simulink model "Finalannfaultdetecandclass"  (R2024b)
settings: Solver=ode45  StartTime=0.0  StopTime=0.4  FixedStep=1e-6  MaxStep=0.04  RelTol=1e-3  EnableMultiTasking=on
PreLoadFcn:
  | power_13NodeTestFeeder_init;
values from neighbouring files (symbols this model uses):
  C_601 = [1.03835973183e-08  -3.28956213337e-09  -2.07596127216e-09; -3.28956213337e-09  9.8230300863e-09  -1.22250137004e-09; -2.07596127216e-09  -1.22250137004e-09  9.29377945947e-09]    [Finalmat.mat]    (also in bus1.mat; bus10.mat; bus11.mat; bus12.mat)
  C_602 = [9.39333329896e-09  -1.78290377777e-09  -2.78635373607e-09; -1.78290377777e-09  8.5370713848e-09  -1.08586207709e-09; -2.78635373607e-09  -1.08586207709e-09  8.94105559107e-09]    [Finalmat.mat]    (also in bus1.mat; bus10.mat; bus11.mat; bus12.mat)
  C_603 = [0  0  0; 0  7.76272711671e-09  -1.48325331387e-09; 0  -1.48325331387e-09  7.69036927641e-09]    [Finalmat.mat]    (also in bus1.mat; bus10.mat; bus11.mat; bus12.mat)
  C_604 = [7.69036927641e-09  0  -1.48325331387e-09; 0  0  0; -1.48325331387e-09  0  7.76272711671e-09]    [Finalmat.mat]    (also in bus1.mat; bus10.mat; bus11.mat; bus12.mat)
  C_605 = [0  0  0; 0  0  0; 0  0  7.44890176838e-09]    [Finalmat.mat]    (also in bus1.mat; bus10.mat; bus11.mat; bus12.mat)
  C_606 = [1.59697709306e-07  -1.64824237567e-15  -1.64824237567e-15; -1.64824237567e-15  1.59697709306e-07  -1.64824237567e-15; -1.64824237567e-15  -1.64824237567e-15  1.59697709306e-07]    [Finalmat.mat]    (also in bus1.mat; bus10.mat; bus11.mat; bus12.mat)
  C_607 = [1.46679066902e-07  0  0; 0  0  0; 0  0  0]    [Finalmat.mat]    (also in bus1.mat; bus10.mat; bus11.mat; bus12.mat)
  ft2km = 0.0003048    [Finalmat.mat]    (also in bus1.mat; bus10.mat; bus11.mat; bus12.mat)
  L_601 = [0.0016777459142  0.000826923199875  0.000698195470335; 0.000826923199875  0.00172702836123  0.000634408490396; 0.000698195470335  0.000634408490396  0.00170560121035]    [Finalmat.mat]    (also in bus1.mat; bus10.mat; bus11.mat; bus12.mat)
  L_602 = [0.00194723354262  0.000698195470335  0.000826923199875; 0.000698195470335  0.00197508883877  0.000634408490396; 0.000826923199875  0.000634408490396  0.00199635116541]    [Finalmat.mat]    (also in bus1.mat; bus10.mat; bus11.mat; bus12.mat)
  L_603 = [0  0  0; 0  0.00222034730427  0.000756708074671; 0  0.000756708074671  0.00223650007955]    [Finalmat.mat]    (also in bus1.mat; bus10.mat; bus11.mat; bus12.mat)
  L_604 = [0.00223650007955  0  0.000756708074671; 0  0  0; 0.000756708074671  0  0.00222034730427]    [Finalmat.mat]    (also in bus1.mat; bus10.mat; bus11.mat; bus12.mat)
  L_605 = [0  0  0; 0  0  0; 0  0  0.00222100660122]    [Finalmat.mat]    (also in bus1.mat; bus10.mat; bus11.mat; bus12.mat)
  L_606 = [0.000735610572263  5.40623499221e-05  2.35698659721e-05; 5.40623499221e-05  0.000666054744009  5.40623499221e-05; 2.35698659721e-05  5.40623499221e-05  0.000735610572263]    [Finalmat.mat]    (also in bus1.mat; bus10.mat; bus11.mat; bus12.mat)
  L_607 = [0.000844559393295  0  0; 0  0  0; 0  0  0]    [Finalmat.mat]    (also in bus1.mat; bus10.mat; bus11.mat; bus12.mat)
  R_601 = [0.215305653249  0.0969341469174  0.0981768923907; 0.0969341469174  0.209713298619  0.0953807150757; 0.0981768923907  0.0953807150757  0.212136652292]    [Finalmat.mat]    (also in bus1.mat; bus10.mat; bus11.mat; bus12.mat)
  R_602 = [0.467645121603  0.0981768923907  0.0969341469174; 0.0981768923907  0.464476120646  0.0953807150757; 0.0969341469174  0.0953807150757  0.462052766973]    [Finalmat.mat]    (also in bus1.mat; bus10.mat; bus11.mat; bus12.mat)
  R_603 = [0  0  0; 0  0.826052916102  0.128375607392; 0  0.128375607392  0.822573228777]    [Finalmat.mat]    (also in bus1.mat; bus10.mat; bus11.mat; bus12.mat)
  R_604 = [0.822573228777  0  0.128375607392; 0  0  0; 0.128375607392  0  0.826052916102]    [Finalmat.mat]    (also in bus1.mat; bus10.mat; bus11.mat; bus12.mat)
  R_605 = [0  0  0; 0  0  0; 0  0  0.825928641555]    [Finalmat.mat]    (also in bus1.mat; bus10.mat; bus11.mat; bus12.mat)
  R_606 = [0.495979718394  0.198342177539  0.177029092672; 0.198342177539  0.49032522649  0.198342177539; 0.177029092672  0.198342177539  0.495979718394]    [Finalmat.mat]    (also in bus1.mat; bus10.mat; bus11.mat; bus12.mat)
  R_607 = [0.834192898952  0  0; 0  0  0; 0  0  0]    [Finalmat.mat]    (also in bus1.mat; bus10.mat; bus11.mat; bus12.mat)
libraries: neural x123, spsLoadFlowBusLib x12, spsDistributedParametersLineLib x9, spsThreePhaseSeriesRLCLoadLib x7, spsMultimeterLib x6, spsPowerPhasorLib x6, spsSeriesRLCLoadLib x5, spsThreePhaseVIMeasurementLib x4, spsGroundLib x4, spsThreePhaseSourceLib x1, spsThreePhaseBreakerLib x1, simulink x1
(part 4 of 4)

== system Finalannfaultdetecandclass/Subsystem1/Function Fitting Neural Network/Layer 2/Delays 1 ==
  "p{2}" : Inport  PortDimensions=100
      mask Display: e = 0.06;c1 = [120 230 180]/255;c2 = ([120 230 180]+0)/(256+128);c3 = ([120 230 180]+128)/(256+128);patch([0 1 1 0],[0 0 1 1],c1);patch([0 1 1 1-e 1-e 0+e],[0 0 1 1-e 0+e 0+e],c2);patch([0 0 1 1-e 0+e 0+e],[0 1 1 1-e 1-e 0+e],c3);plot([0 1 1 0 0],[0 0 1 1 0]);
  mux : Mux  Inputs=1
      mask Display: e = 0.06;c1 = [120 150 230]/255;c2 = ([120 150 230]+0)/383;c3 = ([120 150 230]+128)/383;patch([0 1 1 0],[0 0 1 1],c1);patch([0 1 1 1-e 1-e 0+e],[0 0 1 1-e 0+e 0+e],c2);patch([0 0 1 1-e 0+e 0+e],[0 1 1 1-e 1-e 0+e],c3);plot([0 1 1 0 0],[0 0 1 1 0]);disp('Mux')
  "pd{2,1}" : Outport
      mask Display: e = 0.06;c1 = [120 230 180]/255;c2 = ([120 230 180]+0)/(256+128);c3 = ([120 230 180]+128)/(256+128);patch([0 1 1 0],[0 0 1 1],c1);patch([0 1 1 1-e 1-e 0+e],[0 0 1 1-e 0+e 0+e],c2);patch([0 0 1 1-e 0+e 0+e],[0 1 1 1-e 1-e 0+e],c3);plot([0 1 1 0 0],[0 0 1 1 0]);
  wires:
  "p{2}"/1 -> mux/1
  mux/1 -> "pd{2,1}"/1

== system Finalannfaultdetecandclass/Subsystem1/Function Fitting Neural Network/Layer 2/LW{2,1} ==
  "ad{2,1}" : Inport  PortDimensions=100
      mask Display: e = 0.06;c1 = [120 230 180]/255;c2 = ([120 230 180]+0)/(256+128);c3 = ([120 230 180]+128)/(256+128);patch([0 1 1 0],[0 0 1 1],c1);patch([0 1 1 1-e 1-e 0+e],[0 0 1 1-e 0+e 0+e],c2);patch([0 0 1 1-e 0+e 0+e],[0 1 1 1-e 1-e 0+e],c3);plot([0 1 1 0 0],[0 0 1 1 0]);
  "IW{2,1}(1,:)'" : Constant  Value=[1.8793908287279783575485225810552947223186492919921875;-0.9048667518245905316831567688495852053165435791015625;-0.92458538808867185565532054170034825801849365234375;-2.02532521067546245063795140595175325870513916015625;5.33525657670273556476558951544575393199920654296875;3.210800612231773154547909143730066716670989990234375;-0.09324484938112427567791229421345633454620838165283203125;0.03540388689183378290170622904042829759418964385986328125;0.1885587765727710640728531643617316149175167083740234375;-4.22107099118371120738402169081382453441619873046875;-0.264501726010362647745211006622412241995334625244140625;-0.34225779722053040199369888796354644000530242919921875;-0.373202417779953388166092054234468378126621246337890625;8.2600182662194896465734927915036678314208984375;-3.2632258813898840088540964643470942974090576171875;-0.62922711116860108315762545316829346120357513427734375;-0.38755461469218255299296060911729000508785247802734375;0.65203344442902988475907477550208568572998046875;-2.26821878466440285393446174566633999347686767578125;0.543177487170682926631570808240212500095367431640625;-2.789913530456374690658094550599344074726104736328125;0.1798698221775162642277479108088300563395023345947265625;0.399305983587987689542586622337694279849529266357421875;1.2306887105144139749057785593322478234767913818359375;1.456708317179773448657442713738419115543365478515625;1.035561461053104093110732719651423394680023193359375;0.27441751827051164003279382086475379765033721923828125;-0.204970973074732831786803899376536719501018524169921875;-0.253112822104407164669481744567747227847576141357421875;0.1510518587617716013138391417669481597840785980224609375;-0.31745069317599250435790736446506343781948089599609375;-0.676791919103845618366221970063634216785430908203125;-2.978627056642336068392751258215866982936859130859375;9.0535751730324189878729157499037683010101318359375;-8.190932561555936075592398992739617824554443359375;0.49841770298888565804418249172158539295196533203125;-0.50061513193962159373739950751769356429576873779296875;1.53295551447780287190880699199624359607696533203125;12.583976878439415258981171064078807830810546875;-0.09178682720573481945702809525755583308637142181396484375;8.636594135212391165623557753860950469970703125;3.910230596444252970655952594825066626071929931640625;-2.50969331155198016602980715106241405010223388671875;-0.32572264372845494140307209818274714052677154541015625;2.658418596062821048775504095829091966152191162109375;4.26885657500254556140362183214165270328521728515625;1.4483077928253802468816502369008958339691162109375;-1.0548868080331390562065507765510119497776031494140625;-1.75700921521880726317021981230936944484710693359375;-4.8518766072740096007009924505837261676788330078125;-0.043810031439321835133871019252183032222092151641845703125;0.418247245768505415686178139367257244884967803955078125;-1.54235777001860352442008661455474793910980224609375;0.2440732320832143809052894312117132358253002166748046875;-2.981478415506142010116263918462209403514862060546875;-0.1983812993079519804151544803971773944795131683349609375;-0.488626450603534212557832461243378929793834686279296875;-4.16709607961305028567267072503454983234405517578125;2.59533520027240083294373107491992413997650146484375;4.20601887646172389878529429552145302295684814453125;3.531120270555935025669214155641384422779083251953125;-0.51904717173316872180777181711164303123950958251953125;1.751606913577048896257792875985614955425262451171875;2.297924274586310655621446130680851638317108154296875;0.10235191318978331675992876625969074666500091552734375;0.68318748611821000782384771810029633343219757080078125;1.0577758447114204987116181655437685549259185791015625;3.15370331022145489185959377209655940532684326171875;1.325141327935329460530056167044676840305328369140625;4.03421651104892742267793437349610030651092529296875;-9.5505906993198106391673718462698161602020263671875;-0.21252767811685158161338904392323456704616546630859375 ...(+1553 chars)]
      mask Display: e = 0.06;c1 = [120 150 230]/255;c2 = ([120 150 230]+0)/383;c3 = ([120 150 230]+128)/383;patch([0 1 1 0],[0 0 1 1],c1);patch([0 1 1 1-e 1-e 0+e],[0 0 1 1-e 0+e 0+e],c2);patch([0 0 1 1-e 0+e 0+e],[0 1 1 1-e 1-e 0+e],c3);plot([0 1 1 0 0],[0 0 1 1 0]);disp('weights');
  Mux : Mux  Inputs=1
      mask Display: e = 0.06;c1 = [120 150 230]/255;c2 = ([120 150 230]+0)/383;c3 = ([120 150 230]+128)/383;patch([0 1 1 0],[0 0 1 1],c1);patch([0 1 1 1-e 1-e 0+e],[0 0 1 1-e 0+e 0+e],c2);patch([0 0 1 1-e 0+e 0+e],[0 1 1 1-e 1-e 0+e],c3);plot([0 1 1 0 0],[0 0 1 1 0]);disp('Mux');
  dotprod1 : neural/Weight Functions/dotprod
  "lz{2,1}" : Outport
      mask Display: e = 0.06;c1 = [120 230 180]/255;c2 = ([120 230 180]+0)/(256+128);c3 = ([120 230 180]+128)/(256+128);patch([0 1 1 0],[0 0 1 1],c1);patch([0 1 1 1-e 1-e 0+e],[0 0 1 1-e 0+e 0+e],c2);patch([0 0 1 1-e 0+e 0+e],[0 1 1 1-e 1-e 0+e],c3);plot([0 1 1 0 0],[0 0 1 1 0]);
  wires:
  "IW{2,1}(1,:)'"/1 -> dotprod1/1
  "ad{2,1}"/1 -> dotprod1/2
  dotprod1/1 -> Mux/1
  Mux/1 -> "lz{2,1}"/1

== system Finalannfaultdetecandclass/Subsystem1/Function Fitting Neural Network1/Layer 1/Delays 1 ==
  "p{1}" : Inport  PortDimensions=9
      mask Display: e = 0.06;c1 = [120 230 180]/255;c2 = ([120 230 180]+0)/(256+128);c3 = ([120 230 180]+128)/(256+128);patch([0 1 1 0],[0 0 1 1],c1);patch([0 1 1 1-e 1-e 0+e],[0 0 1 1-e 0+e 0+e],c2);patch([0 0 1 1-e 0+e 0+e],[0 1 1 1-e 1-e 0+e],c3);plot([0 1 1 0 0],[0 0 1 1 0]);
  mux : Mux  Inputs=1
      mask Display: e = 0.06;c1 = [120 150 230]/255;c2 = ([120 150 230]+0)/383;c3 = ([120 150 230]+128)/383;patch([0 1 1 0],[0 0 1 1],c1);patch([0 1 1 1-e 1-e 0+e],[0 0 1 1-e 0+e 0+e],c2);patch([0 0 1 1-e 0+e 0+e],[0 1 1 1-e 1-e 0+e],c3);plot([0 1 1 0 0],[0 0 1 1 0]);disp('Mux')
  "pd{1,1}" : Outport
      mask Display: e = 0.06;c1 = [120 230 180]/255;c2 = ([120 230 180]+0)/(256+128);c3 = ([120 230 180]+128)/(256+128);patch([0 1 1 0],[0 0 1 1],c1);patch([0 1 1 1-e 1-e 0+e],[0 0 1 1-e 0+e 0+e],c2);patch([0 0 1 1-e 0+e 0+e],[0 1 1 1-e 1-e 0+e],c3);plot([0 1 1 0 0],[0 0 1 1 0]);
  wires:
  "p{1}"/1 -> mux/1
  mux/1 -> "pd{1,1}"/1

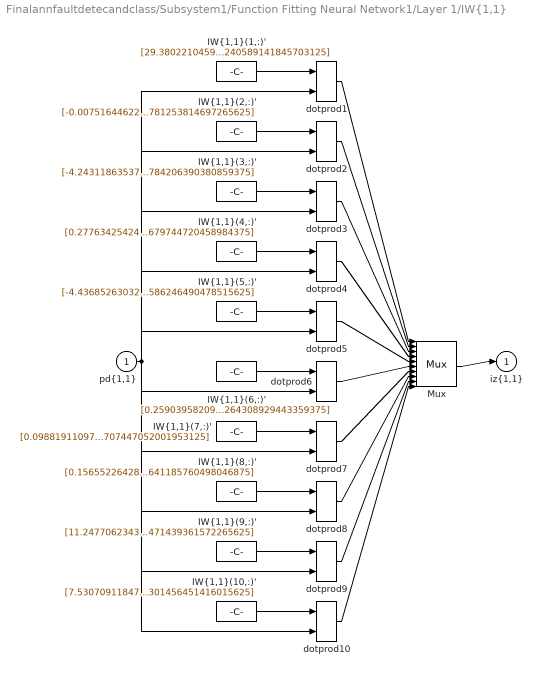
== system Finalannfaultdetecandclass/Subsystem1/Function Fitting Neural Network1/Layer 1/IW{1,1} ==
  "pd{1,1}" : Inport  PortDimensions=9
      mask Display: e = 0.06;c1 = [120 230 180]/255;c2 = ([120 230 180]+0)/(256+128);c3 = ([120 230 180]+128)/(256+128);patch([0 1 1 0],[0 0 1 1],c1);patch([0 1 1 1-e 1-e 0+e],[0 0 1 1-e 0+e 0+e],c2);patch([0 0 1 1-e 0+e 0+e],[0 1 1 1-e 1-e 0+e],c3);plot([0 1 1 0 0],[0 0 1 1 0]);
  "IW{1,1}(1,:)'" : Constant  Value=[29.38022104594626426887771231122314929962158203125;-1.583758512931292106173941647284664213657379150390625;-12.887641563029934133055576239712536334991455078125;15.3742096899572491253138650790788233280181884765625;-0.452999735082487919868299286463297903537750244140625;-11.2742404077810487450506116147153079509735107421875;0.253929560001421028569978943778551183640956878662109375;13.720895642811651526926652877591550350189208984375;3.625389934006417735901095511508174240589141845703125]
      mask Display: e = 0.06;c1 = [120 150 230]/255;c2 = ([120 150 230]+0)/383;c3 = ([120 150 230]+128)/383;patch([0 1 1 0],[0 0 1 1],c1);patch([0 1 1 1-e 1-e 0+e],[0 0 1 1-e 0+e 0+e],c2);patch([0 0 1 1-e 0+e 0+e],[0 1 1 1-e 1-e 0+e],c3);plot([0 1 1 0 0],[0 0 1 1 0]);disp('Weights');
  "IW{1,1}(10,:)'" : Constant  Value=[7.530709118478295494014673749916255474090576171875;6.41481450944031461602889976347796618938446044921875;5.7414808644690840111479701590724289417266845703125;-1.0144361351505650770121746973018161952495574951171875;0.60391139595748588586587857207632623612880706787109375;0.175120384899493497510292172592016868293285369873046875;-6.341914830455859686253461404703557491302490234375;1.329104495916630934715385592426173388957977294921875;4.685489713819865897903582663275301456451416015625]
      mask Display: e = 0.06;c1 = [120 150 230]/255;c2 = ([120 150 230]+0)/383;c3 = ([120 150 230]+128)/383;patch([0 1 1 0],[0 0 1 1],c1);patch([0 1 1 1-e 1-e 0+e],[0 0 1 1-e 0+e 0+e],c2);patch([0 0 1 1-e 0+e 0+e],[0 1 1 1-e 1-e 0+e],c3);plot([0 1 1 0 0],[0 0 1 1 0]);disp('Weights');
  "IW{1,1}(2,:)'" : Constant  Value=[-0.007516446226203031544255139806409715674817562103271484375;-0.052171455998463005243603873850588570348918437957763671875;40.07240766673493226335267536342144012451171875;-0.529361813414303217228962239460088312625885009765625;-0.1313103612760208316334598066532635129988193511962890625;0.492305801062109138488409598721773363649845123291015625;-0.2409650475170437566863057554655824787914752960205078125;-9.543939777753767117474126280285418033599853515625;9.0870090560286005398893394158221781253814697265625]
      mask Display: e = 0.06;c1 = [120 150 230]/255;c2 = ([120 150 230]+0)/383;c3 = ([120 150 230]+128)/383;patch([0 1 1 0],[0 0 1 1],c1);patch([0 1 1 1-e 1-e 0+e],[0 0 1 1-e 0+e 0+e],c2);patch([0 0 1 1-e 0+e 0+e],[0 1 1 1-e 1-e 0+e],c3);plot([0 1 1 0 0],[0 0 1 1 0]);disp('Weights');
  "IW{1,1}(3,:)'" : Constant  Value=[-4.24311863537578748406531303771771490573883056640625;-0.56605455006675431395279929347452707588672637939453125;7.69263762371459502986681400216184556484222412109375;-0.2345349318144732964075416248306282795965671539306640625;0.43859983264558854987313907258794642984867095947265625;0.72900485968290917870859857430332340300083160400390625;-0.6106674688833038100455041785608045756816864013671875;-1.4125342046991329336691478602006100118160247802734375;0.954529878403048481771975275478325784206390380859375]
      mask Display: e = 0.06;c1 = [120 150 230]/255;c2 = ([120 150 230]+0)/383;c3 = ([120 150 230]+128)/383;patch([0 1 1 0],[0 0 1 1],c1);patch([0 1 1 1-e 1-e 0+e],[0 0 1 1-e 0+e 0+e],c2);patch([0 0 1 1-e 0+e 0+e],[0 1 1 1-e 1-e 0+e],c3);plot([0 1 1 0 0],[0 0 1 1 0]);disp('Weights');
  "IW{1,1}(4,:)'" : Constant  Value=[0.27763425424716647871292707350221462547779083251953125;-3.3827539479368713415396996424533426761627197265625;-0.487081651909694601787492729272344149649143218994140625;-6.9426781475629635309587683877907693386077880859375;0.2001253526836813956268912306768470443785190582275390625;-0.321497490473505731500836191116832196712493896484375;-12.4322080410378870141130391857586801052093505859375;12.5879994895972320279042833135463297367095947265625;0.27710769892183806373253673882572911679744720458984375]
      mask Display: e = 0.06;c1 = [120 150 230]/255;c2 = ([120 150 230]+0)/383;c3 = ([120 150 230]+128)/383;patch([0 1 1 0],[0 0 1 1],c1);patch([0 1 1 1-e 1-e 0+e],[0 0 1 1-e 0+e 0+e],c2);patch([0 0 1 1-e 0+e 0+e],[0 1 1 1-e 1-e 0+e],c3);plot([0 1 1 0 0],[0 0 1 1 0]);disp('Weights');
  "IW{1,1}(5,:)'" : Constant  Value=[-4.4368526303241448971448335214518010616302490234375;-3.593845053872443795484059592126868665218353271484375;10.1550055068302498284538160078227519989013671875;-0.49914763675904272322014776364085264503955841064453125;0.5660702345538994872953253434388898313045501708984375;1.37378804025246825659678506781347095966339111328125;-0.405236667080652368522208917056559585034847259521484375;-1.4087649953617231712854618308483622968196868896484375;1.5632128167424907960736391032696701586246490478515625]
      mask Display: e = 0.06;c1 = [120 150 230]/255;c2 = ([120 150 230]+0)/383;c3 = ([120 150 230]+128)/383;patch([0 1 1 0],[0 0 1 1],c1);patch([0 1 1 1-e 1-e 0+e],[0 0 1 1-e 0+e 0+e],c2);patch([0 0 1 1-e 0+e 0+e],[0 1 1 1-e 1-e 0+e],c3);plot([0 1 1 0 0],[0 0 1 1 0]);disp('Weights');
  "IW{1,1}(6,:)'" : Constant  Value=[0.25903958209407884627495377571904100477695465087890625;-14.1728596158761632750611170195043087005615234375;13.9842637333953359046745390514843165874481201171875;-0.18984682930795060418205366659094579517841339111328125;-0.3858122437420750117098577902652323246002197265625;0.66984843931265292127363863983191549777984619140625;-4.72065980238203319885315067949704825878143310546875;5.22961841369345581398420108598656952381134033203125;3.5168686234222885644840062013827264308929443359375]
      mask Display: e = 0.06;c1 = [120 150 230]/255;c2 = ([120 150 230]+0)/383;c3 = ([120 150 230]+128)/383;patch([0 1 1 0],[0 0 1 1],c1);patch([0 1 1 1-e 1-e 0+e],[0 0 1 1-e 0+e 0+e],c2);patch([0 0 1 1-e 0+e 0+e],[0 1 1 1-e 1-e 0+e],c3);plot([0 1 1 0 0],[0 0 1 1 0]);disp('Weights');
  "IW{1,1}(7,:)'" : Constant  Value=[0.0988191109786849819496268310103914700448513031005859375;29.522862844008496807646224624477326869964599609375;0.4973642899908086167926057896693237125873565673828125;-7.157403678754118203642065054737031459808349609375;9.3605112948433220054766934481449425220489501953125;-0.4133008665678818971400687587447464466094970703125;-22.339928592137457741273465217091143131256103515625;-4.193358410228416488507718895561993122100830078125;-2.057182487229031853104288529721088707447052001953125]
      mask Display: e = 0.06;c1 = [120 150 230]/255;c2 = ([120 150 230]+0)/383;c3 = ([120 150 230]+128)/383;patch([0 1 1 0],[0 0 1 1],c1);patch([0 1 1 1-e 1-e 0+e],[0 0 1 1-e 0+e 0+e],c2);patch([0 0 1 1-e 0+e 0+e],[0 1 1 1-e 1-e 0+e],c3);plot([0 1 1 0 0],[0 0 1 1 0]);disp('Weights');
  "IW{1,1}(8,:)'" : Constant  Value=[0.1565522642874812297986153453166480176150798797607421875;0.07335552424086433376260174554772675037384033203125;0.493599606767612775204412400853470899164676666259765625;-2.575576222935119563572925471817143261432647705078125;-5.204489703361520724911315483041107654571533203125;-1.495166781266143107842481185798533260822296142578125;-0.30736378638011974118171565351076424121856689453125;-24.3238565177839376474366872571408748626708984375;0.9721005384518004444061034519108943641185760498046875]
      mask Display: e = 0.06;c1 = [120 150 230]/255;c2 = ([120 150 230]+0)/383;c3 = ([120 150 230]+128)/383;patch([0 1 1 0],[0 0 1 1],c1);patch([0 1 1 1-e 1-e 0+e],[0 0 1 1-e 0+e 0+e],c2);patch([0 0 1 1-e 0+e 0+e],[0 1 1 1-e 1-e 0+e],c3);plot([0 1 1 0 0],[0 0 1 1 0]);disp('Weights');
  "IW{1,1}(9,:)'" : Constant  Value=[11.2477062343173290770437233732081949710845947265625;0.01906889569289538233221037444309331476688385009765625;3.306004742964588682951898590545170009136199951171875;-0.4465209024047254171563281488488428294658660888671875;-0.154686319042484476948828842068905942142009735107421875;-0.039328003291225162307842566633553360588848590850830078125;0.1089866231528095752434381893181125633418560028076171875;-6.49190528631474439436033208039589226245880126953125;5.89332989152609432181861848221160471439361572265625]
      mask Display: e = 0.06;c1 = [120 150 230]/255;c2 = ([120 150 230]+0)/383;c3 = ([120 150 230]+128)/383;patch([0 1 1 0],[0 0 1 1],c1);patch([0 1 1 1-e 1-e 0+e],[0 0 1 1-e 0+e 0+e],c2);patch([0 0 1 1-e 0+e 0+e],[0 1 1 1-e 1-e 0+e],c3);plot([0 1 1 0 0],[0 0 1 1 0]);disp('Weights');
  Mux : Mux  Inputs=10
      mask Display: e = 0.06;c1 = [120 150 230]/255;c2 = ([120 150 230]+0)/383;c3 = ([120 150 230]+128)/383;patch([0 1 1 0],[0 0 1 1],c1);patch([0 1 1 1-e 1-e 0+e],[0 0 1 1-e 0+e 0+e],c2);patch([0 0 1 1-e 0+e 0+e],[0 1 1 1-e 1-e 0+e],c3);plot([0 1 1 0 0],[0 0 1 1 0]);disp('Mux');
  dotprod{1..10} (10 alike) : neural/Weight Functions/dotprod
  "iz{1,1}" : Outport
      mask Display: e = 0.06;c1 = [120 230 180]/255;c2 = ([120 230 180]+0)/(256+128);c3 = ([120 230 180]+128)/(256+128);patch([0 1 1 0],[0 0 1 1],c1);patch([0 1 1 1-e 1-e 0+e],[0 0 1 1-e 0+e 0+e],c2);patch([0 0 1 1-e 0+e 0+e],[0 1 1 1-e 1-e 0+e],c3);plot([0 1 1 0 0],[0 0 1 1 0]);
  wires:
  "IW{1,1}(1,:)'"/1 -> dotprod1/1
  "pd{1,1}"/1 -> dotprod1/2, dotprod2/2, dotprod3/2, dotprod4/2, dotprod5/2, dotprod6/2, dotprod7/2, dotprod8/2, dotprod9/2, dotprod10/2
  dotprod1/1 -> Mux/1
  "IW{1,1}(2,:)'"/1 -> dotprod2/1
  dotprod2/1 -> Mux/2
  "IW{1,1}(3,:)'"/1 -> dotprod3/1
  dotprod3/1 -> Mux/3
  "IW{1,1}(4,:)'"/1 -> dotprod4/1
  dotprod4/1 -> Mux/4
  "IW{1,1}(5,:)'"/1 -> dotprod5/1
  dotprod5/1 -> Mux/5
  "IW{1,1}(6,:)'"/1 -> dotprod6/1
  dotprod6/1 -> Mux/6
  "IW{1,1}(7,:)'"/1 -> dotprod7/1
  dotprod7/1 -> Mux/7
  "IW{1,1}(8,:)'"/1 -> dotprod8/1
  dotprod8/1 -> Mux/8
  "IW{1,1}(9,:)'"/1 -> dotprod9/1
  dotprod9/1 -> Mux/9
  "IW{1,1}(10,:)'"/1 -> dotprod10/1
  dotprod10/1 -> Mux/10
  Mux/1 -> "iz{1,1}"/1

== system Finalannfaultdetecandclass/Subsystem1/Function Fitting Neural Network1/Layer 2/Delays 1 ==
  "p{2}" : Inport  PortDimensions=10
      mask Display: e = 0.06;c1 = [120 230 180]/255;c2 = ([120 230 180]+0)/(256+128);c3 = ([120 230 180]+128)/(256+128);patch([0 1 1 0],[0 0 1 1],c1);patch([0 1 1 1-e 1-e 0+e],[0 0 1 1-e 0+e 0+e],c2);patch([0 0 1 1-e 0+e 0+e],[0 1 1 1-e 1-e 0+e],c3);plot([0 1 1 0 0],[0 0 1 1 0]);
  mux : Mux  Inputs=1
      mask Display: e = 0.06;c1 = [120 150 230]/255;c2 = ([120 150 230]+0)/383;c3 = ([120 150 230]+128)/383;patch([0 1 1 0],[0 0 1 1],c1);patch([0 1 1 1-e 1-e 0+e],[0 0 1 1-e 0+e 0+e],c2);patch([0 0 1 1-e 0+e 0+e],[0 1 1 1-e 1-e 0+e],c3);plot([0 1 1 0 0],[0 0 1 1 0]);disp('Mux')
  "pd{2,1}" : Outport
      mask Display: e = 0.06;c1 = [120 230 180]/255;c2 = ([120 230 180]+0)/(256+128);c3 = ([120 230 180]+128)/(256+128);patch([0 1 1 0],[0 0 1 1],c1);patch([0 1 1 1-e 1-e 0+e],[0 0 1 1-e 0+e 0+e],c2);patch([0 0 1 1-e 0+e 0+e],[0 1 1 1-e 1-e 0+e],c3);plot([0 1 1 0 0],[0 0 1 1 0]);
  wires:
  "p{2}"/1 -> mux/1
  mux/1 -> "pd{2,1}"/1

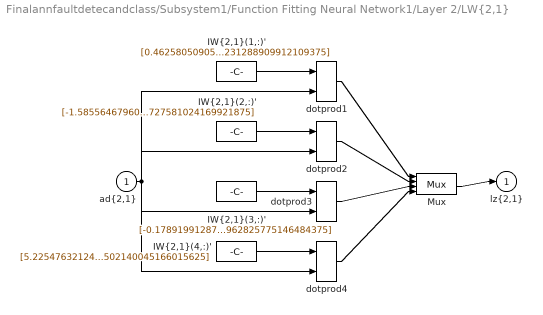
== system Finalannfaultdetecandclass/Subsystem1/Function Fitting Neural Network1/Layer 2/LW{2,1} ==
  "ad{2,1}" : Inport  PortDimensions=10
      mask Display: e = 0.06;c1 = [120 230 180]/255;c2 = ([120 230 180]+0)/(256+128);c3 = ([120 230 180]+128)/(256+128);patch([0 1 1 0],[0 0 1 1],c1);patch([0 1 1 1-e 1-e 0+e],[0 0 1 1-e 0+e 0+e],c2);patch([0 0 1 1-e 0+e 0+e],[0 1 1 1-e 1-e 0+e],c3);plot([0 1 1 0 0],[0 0 1 1 0]);
  "IW{2,1}(1,:)'" : Constant  Value=[0.46258050905511038930484346565208397805690765380859375;-0.491318793492770689024240482467575930058956146240234375;2.600772456187484760192774047027342021465301513671875;2.66426961059672162690503682824783027172088623046875;-3.8671995563505703330520191229879856109619140625;3.072577355630674134090440929867327213287353515625;2.686487956136232480019998547504656016826629638671875;-0.295675430718155052289830564404837787151336669921875;3.914768549273121234222116981982253491878509521484375;-4.5054014070964054639034657157026231288909912109375]
      mask Display: e = 0.06;c1 = [120 150 230]/255;c2 = ([120 150 230]+0)/383;c3 = ([120 150 230]+128)/383;patch([0 1 1 0],[0 0 1 1],c1);patch([0 1 1 1-e 1-e 0+e],[0 0 1 1-e 0+e 0+e],c2);patch([0 0 1 1-e 0+e 0+e],[0 1 1 1-e 1-e 0+e],c3);plot([0 1 1 0 0],[0 0 1 1 0]);disp('weights');
  "IW{2,1}(2,:)'" : Constant  Value=[-1.58556467960289015906027998425997793674468994140625;-0.54767254618767158280689955063280649483203887939453125;-10.7777906158480885068229326861910521984100341796875;-5.19679680077603567411870244541205465793609619140625;8.4277239442383109491174764116294682025909423828125;0.81550554679807596425433757758582942187786102294921875;0.56233367679444146158829198611783795058727264404296875;7.06809248725992222972536183078773319721221923828125;-3.64262105372553879334418525104410946369171142578125;3.43240893002770075526086657191626727581024169921875]
      mask Display: e = 0.06;c1 = [120 150 230]/255;c2 = ([120 150 230]+0)/383;c3 = ([120 150 230]+128)/383;patch([0 1 1 0],[0 0 1 1],c1);patch([0 1 1 1-e 1-e 0+e],[0 0 1 1-e 0+e 0+e],c2);patch([0 0 1 1-e 0+e 0+e],[0 1 1 1-e 1-e 0+e],c3);plot([0 1 1 0 0],[0 0 1 1 0]);disp('weights');
  "IW{2,1}(3,:)'" : Constant  Value=[-0.178919912879987375031731744456919841468334197998046875;1.247926710614366552221099482267163693904876708984375;-1.4662664506978526635094794983160682022571563720703125;-0.81924181188969880107464405227801762521266937255859375;1.1847903805771247132128110024495981633663177490234375;0.655962945361181493098001737962476909160614013671875;0.2255658656909705073179139844796736724674701690673828125;0.90964304667748507871039009842206723988056182861328125;-0.77112055117324562747427307840553112328052520751953125;0.1102976597492469623684741009128629229962825775146484375]
      mask Display: e = 0.06;c1 = [120 150 230]/255;c2 = ([120 150 230]+0)/383;c3 = ([120 150 230]+128)/383;patch([0 1 1 0],[0 0 1 1],c1);patch([0 1 1 1-e 1-e 0+e],[0 0 1 1-e 0+e 0+e],c2);patch([0 0 1 1-e 0+e 0+e],[0 1 1 1-e 1-e 0+e],c3);plot([0 1 1 0 0],[0 0 1 1 0]);disp('weights');
  "IW{2,1}(4,:)'" : Constant  Value=[5.22547632124793803853890494792722165584564208984375;4.59767499962608194863378230365924537181854248046875;30.72925365079600368289902689866721630096435546875;17.53812890540944380290966364555060863494873046875;-24.007257463950981701827913639135658740997314453125;-6.02512235382848881926065587322227656841278076171875;-1.0807050207900801286342584717203862965106964111328125;-18.04133347846309476381065906025469303131103515625;5.9709631066566171142540042637847363948822021484375;-8.5746877523003863785788780660368502140045166015625]
      mask Display: e = 0.06;c1 = [120 150 230]/255;c2 = ([120 150 230]+0)/383;c3 = ([120 150 230]+128)/383;patch([0 1 1 0],[0 0 1 1],c1);patch([0 1 1 1-e 1-e 0+e],[0 0 1 1-e 0+e 0+e],c2);patch([0 0 1 1-e 0+e 0+e],[0 1 1 1-e 1-e 0+e],c3);plot([0 1 1 0 0],[0 0 1 1 0]);disp('weights');
  Mux : Mux
      mask Display: e = 0.06;c1 = [120 150 230]/255;c2 = ([120 150 230]+0)/383;c3 = ([120 150 230]+128)/383;patch([0 1 1 0],[0 0 1 1],c1);patch([0 1 1 1-e 1-e 0+e],[0 0 1 1-e 0+e 0+e],c2);patch([0 0 1 1-e 0+e 0+e],[0 1 1 1-e 1-e 0+e],c3);plot([0 1 1 0 0],[0 0 1 1 0]);disp('Mux');
  dotprod{1..4} (4 alike) : neural/Weight Functions/dotprod
  "lz{2,1}" : Outport
      mask Display: e = 0.06;c1 = [120 230 180]/255;c2 = ([120 230 180]+0)/(256+128);c3 = ([120 230 180]+128)/(256+128);patch([0 1 1 0],[0 0 1 1],c1);patch([0 1 1 1-e 1-e 0+e],[0 0 1 1-e 0+e 0+e],c2);patch([0 0 1 1-e 0+e 0+e],[0 1 1 1-e 1-e 0+e],c3);plot([0 1 1 0 0],[0 0 1 1 0]);
  wires:
  "IW{2,1}(1,:)'"/1 -> dotprod1/1
  "ad{2,1}"/1 -> dotprod1/2, dotprod2/2, dotprod3/2, dotprod4/2
  dotprod1/1 -> Mux/1
  "IW{2,1}(2,:)'"/1 -> dotprod2/1
  dotprod2/1 -> Mux/2
  "IW{2,1}(3,:)'"/1 -> dotprod3/1
  dotprod3/1 -> Mux/3
  "IW{2,1}(4,:)'"/1 -> dotprod4/1
  dotprod4/1 -> Mux/4
  Mux/1 -> "lz{2,1}"/1
